simulink model "r2_b16a4x64f"  (R2012b)
settings: Solver=VariableStepDiscrete  SolverMode=SingleTasking  StartTime=0.0  StopTime=1  RelTol=1e-3
undefined symbols (not defined in the file): fft_stages, n_bits_ants, n_bits_xengs
libraries: xbsIndex_r4 x26846, casper_library_misc x230, xbsReplacements_r4 x24, casper_library_delays x8, xps_library x5, casper_library_communications x4
(part 51 of 227)

== system r2_b16a4x64f/sys2/tl_reord_flags ==
  note: Time has come
  note: Pulse as
      | value
      | changes
  note: Load value when armed
      | and time has come
      | or loading now
  rst : Inport
  current_time : Inport  Port=2
  load_value : Inport  Port=3
  en : Inport  Port=4
  misci : Inport  Port=5
  Assert : xbsIndex_r4/Assert  assert_type=on  type_source=Explicitly  gui_display_data_type=Fixed-point  arith_type=Boolean  n_bits=16  bin_pt=14  preci_type=Single  exp_width=8  frac_width=24  assert_rate=on  rate_source=Explicitly  period=1  output_port=on  block_type=assert
      settings: block_version=11.4
  Concat9 : xbsIndex_r4/Concat  num_inputs=2  dbl_ovrd=off  block_type=concat
      settings: block_version=10.1.3
  Constant29 : Constant  Value=20
  Delay{1..10,13..14,17..20,25..27} (19 alike) : xbsIndex_r4/Delay  rst=off  infoeditControl=Selection of Reset will increase slice count due to use of real FFs and instead of SRLs  en=off  latency=1  dbl_ovrd=off  reg_retiming=on  block_type=delay
  Delay{11..12,15..16} (4 alike) : xbsIndex_r4/Delay  rst=off  infoeditControl=Selection of Reset will increase slice count due to use of real FFs and instead of SRLs  en=on  latency=1  dbl_ovrd=off  reg_retiming=on  block_type=delay
  Inverter : xbsIndex_r4/Inverter  en=off  latency=0  dbl_ovrd=off  block_type=inv
      settings: block_version=11.4
  Logical1 : xbsIndex_r4/Logical  logical_function=AND  inputs=3  en=off  latency=0  precision=Full  arith_type=Unsigned  n_bits=16  bin_pt=0  align_bp=on  dbl_ovrd=off  block_type=logical
  Logical2 : xbsIndex_r4/Logical  logical_function=OR  inputs=2  en=off  latency=1  precision=Full  arith_type=Unsigned  n_bits=16  bin_pt=0  align_bp=on  dbl_ovrd=off  block_type=logical
  Logical3 : xbsIndex_r4/Logical  logical_function=AND  inputs=2  en=off  latency=0  precision=Full  arith_type=Unsigned  n_bits=16  bin_pt=0  align_bp=on  dbl_ovrd=off  block_type=logical
  Logical4 : xbsIndex_r4/Logical  logical_function=AND  inputs=2  en=off  latency=0  precision=Full  arith_type=Unsigned  n_bits=16  bin_pt=0  align_bp=on  dbl_ovrd=off  block_type=logical
  Logical5 : xbsIndex_r4/Logical  logical_function=OR  inputs=2  en=off  latency=0  precision=Full  arith_type=Unsigned  n_bits=16  bin_pt=0  align_bp=on  dbl_ovrd=off  block_type=logical
  Relational : xbsIndex_r4/Relational  mode=a=b  en=off  latency=1  dbl_ovrd=off  block_type=relational
      settings: block_version=10.1.3
  Slice1 : xbsIndex_r4/Slice  nbits=n_bits_time - n_bits_offset  boolean_output=off  mode=Lower Bit Location + Width  bit1=0  base1=MSB of Input  bit0=n_bits_offset  base0=LSB of Input  dbl_ovrd=off  block_type=slice
  Slice2 : xbsIndex_r4/Slice  nbits=n_bits_time - n_bits_offset  boolean_output=off  mode=Lower Bit Location + Width  bit1=0  base1=MSB of Input  bit0=n_bits_offset  base0=LSB of Input  dbl_ovrd=off  block_type=slice
  control : Subsystem  Tag=xps:sw_reg  AncestorBlock=xps_library/software register  mask(swreg){mode=one value, io_dir=From Processor, io_delay=0, sample_period=1, names=load_time_lsw, bitwidths=32, arith_types=0, bin_pts=0, sim_port=on, show_format=off}
      mask prompts: io_dir "I/O direction"; io_delay "I/O delay"; sample_period "Sample period"; names "Name:"; bitwidths "Bitwidth:"; arith_types "Type (ufix=0, fix=1, bool=2):"; bin_pts "Binary pt:"; sim_port "Provide sim input/output?"; show_format "Print format string?"
      mask init:
      | swreg_init(gcb)
      settings: AttributesFormatString=1input
      mask TypeOptions mode: one value | fields of equal size | fields of arbitrary size
      mask Callback mode: swreg_cb(gcb);
      mask TypeOptions io_dir: To Processor | From Processor
      mask Callback io_dir:
      | mask_enables = get_param(gcb, 'MaskEnables');
      | mask_names = get_param(gcb, 'MaskNames');
      | if strcmp(get_param(gcb, 'io_dir'), 'To Processor'),
      |     mask_enables{ismember(mask_names, 'sample_period')} = 'off';
      | else
      |     mask_enables{ismember(mask_names, 'sample_period')} = 'on';
      | end
      | set_param(gcb, 'MaskEnables', mask_enables);
      mask Callback bitwidths:
      | swreg_maskcheck(gcb);
      | % blk = gcb;
      | % mode = get_param(blk, 'mode');
      | % current_widths = eval(get_param(blk, 'bitwidths'));
      | % if (strcmp(mode, 'one value') || strcmp(mode, 'fields of equal size')) && (length(current_widths) > 1),
      | %     error('Only one width may be specified for this mode.');
      | % elseif strcmp(mode, 'fields of arbitrary size')
      | %     current_names = textscan(strtrim(strrep(strrep(get_param(blk, 'names'), ']', ''), '[', '')), '%s');
      | %     current_names = current_names{1};
      | %     numios = length(current_names);
      | %     if length(current_widths) ~= numios,
      | %         error('%d field names specified, but %d widths?', numios, length(current_widths));
      | %     end
      | % end
      | % total_width = 0;
      | % for ctr = 1 : length(current_widths),
      | %     total_width = total_width + current_widths(ctr);
      | % end
      | % if total_width > 32,
      | %     error('Total width must be 32 or less, set to %d.', total_width);
      | % end
      mask Callback arith_types:
      | [numios, ~, ~, ~, current_types] = swreg_maskcheck(gcb);
      | % blk = gcb;
      | % mode = get_param(blk, 'mode');
      | % current_types = eval(get_param(blk, 'arith_types'));
      | % numios = length(current_types);
      | % if (strcmp(mode, 'one value') || strcmp(mode, 'fields of equal size')) && (length(current_types) > 1),
      | %     error('Only one type may be specified for this mode.');
      | % elseif strcmp(mode, 'fields of arbitrary size')
      | %     current_names = textscan(strtrim(strrep(strrep(get_param(blk, 'names'), ']', ''), '[', '')), '%s');
      | %     current_names = current_names{1};
      | %     numios = length(current_names);
      | %     if length(current_types) ~= numios,
      | %         error('%d field names specified, but %d types?', numios, length(current_types));
      | %     end
      | % end
      | problem = 0;
      | for ctr = 1 : numios,
      |     t = current_types(ctr);
      |     if (t < 0) || (t > 2),
      |         problem = t;
      |         ctr = numios + 1;
      |     end
      | end
      | if problem ~= 0,
      |     error('Type cannot be %i, must be 0, 1 or 2.', problem);
      | end
      mask Callback bin_pts:
      | swreg_maskcheck(gcb);
      | % blk = gcb;
      | % mode = get_param(blk, 'mode');
      | % current_bins = eval(get_param(blk, 'bin_pts'));
      | % if (strcmp(mode, 'one value') || strcmp(mode, 'fields of equal size')) && (length(current_bins) > 1),
      | %     error('Only one binary pt may be specified for this mode.');
      | % elseif strcmp(mode, 'fields of arbitrary size')
      | %     current_names = textscan(strtrim(strrep(strrep(get_param(blk, 'names'), ']', ''), '[', '')), '%s');
      | %     current_names = current_names{1};
      | %     numios = length(current_names);
      | %     if length(current_bins) ~= numios,
      | %         error('%d field names specified, but %d binary pts?', numios, length(current_bins));
      | %     end
      | % end
  control0 : Subsystem  Tag=xps:sw_reg  AncestorBlock=xps_library/software register  mask(swreg){mode=fields of arbitrary size, io_dir=From Processor, io_delay=0, sample_period=1, names=[arm load_immediate load_time_msw], bitwidths=[1 1 16], arith_types=[2 2 0], bin_pts=[0 0 0], sim_port=off, show_format=off}
      mask prompts: io_dir "I/O direction"; io_delay "I/O delay"; sample_period "Sample period"; names "Names [msb ... lsb]:"; bitwidths "Bitwidths [msb ... lsb]:"; arith_types "Types (ufix=0, fix=1, bool=2) [msb ... lsb]:"; bin_pts "Binary pts [msb ... lsb]:"; sim_port "Provide sim input/output?"; show_format "Print format string?"
      mask init:
      | swreg_init(gcb)
      settings: AttributesFormatString=3 inputs
      mask TypeOptions mode: one value | fields of equal size | fields of arbitrary size
      mask Callback mode: swreg_cb(gcb);
      mask TypeOptions io_dir: To Processor | From Processor
      mask Callback io_dir:
      | mask_enables = get_param(gcb, 'MaskEnables');
      | mask_names = get_param(gcb, 'MaskNames');
      | if strcmp(get_param(gcb, 'io_dir'), 'To Processor'),
      |     mask_enables{ismember(mask_names, 'sample_period')} = 'off';
      | else
      |     mask_enables{ismember(mask_names, 'sample_period')} = 'on';
      | end
      | set_param(gcb, 'MaskEnables', mask_enables);
      mask Callback bitwidths:
      | swreg_maskcheck(gcb);
      | % blk = gcb;
      | % mode = get_param(blk, 'mode');
      | % current_widths = eval(get_param(blk, 'bitwidths'));
      | % if (strcmp(mode, 'one value') || strcmp(mode, 'fields of equal size')) && (length(current_widths) > 1),
      | %     error('Only one width may be specified for this mode.');
      | % elseif strcmp(mode, 'fields of arbitrary size')
      | %     current_names = textscan(strtrim(strrep(strrep(get_param(blk, 'names'), ']', ''), '[', '')), '%s');
      | %     current_names = current_names{1};
      | %     numios = length(current_names);
      | %     if length(current_widths) ~= numios,
      | %         error('%d field names specified, but %d widths?', numios, length(current_widths));
      | %     end
      | % end
      | % total_width = 0;
      | % for ctr = 1 : length(current_widths),
      | %     total_width = total_width + current_widths(ctr);
      | % end
      | % if total_width > 32,
      | %     error('Total width must be 32 or less, set to %d.', total_width);
      | % end
      mask Callback arith_types:
      | [numios, ~, ~, ~, current_types] = swreg_maskcheck(gcb);
      | % blk = gcb;
      | % mode = get_param(blk, 'mode');
      | % current_types = eval(get_param(blk, 'arith_types'));
      | % numios = length(current_types);
      | % if (strcmp(mode, 'one value') || strcmp(mode, 'fields of equal size')) && (length(current_types) > 1),
      | %     error('Only one type may be specified for this mode.');
      | % elseif strcmp(mode, 'fields of arbitrary size')
      | %     current_names = textscan(strtrim(strrep(strrep(get_param(blk, 'names'), ']', ''), '[', '')), '%s');
      | %     current_names = current_names{1};
      | %     numios = length(current_names);
      | %     if length(current_types) ~= numios,
      | %         error('%d field names specified, but %d types?', numios, length(current_types));
      | %     end
      | % end
      | problem = 0;
      | for ctr = 1 : numios,
      |     t = current_types(ctr);
      |     if (t < 0) || (t > 2),
      |         problem = t;
      |         ctr = numios + 1;
      |     end
      | end
      | if problem ~= 0,
      |     error('Type cannot be %i, must be 0, 1 or 2.', problem);
      | end
      mask Callback bin_pts:
      | swreg_maskcheck(gcb);
      | % blk = gcb;
      | % mode = get_param(blk, 'mode');
      | % current_bins = eval(get_param(blk, 'bin_pts'));
      | % if (strcmp(mode, 'one value') || strcmp(mode, 'fields of equal size')) && (length(current_bins) > 1),
      | %     error('Only one binary pt may be specified for this mode.');
      | % elseif strcmp(mode, 'fields of arbitrary size')
      | %     current_names = textscan(strtrim(strrep(strrep(get_param(blk, 'names'), ']', ''), '[', '')), '%s');
      | %     current_names = current_names{1};
      | %     numios = length(current_names);
      | %     if length(current_bins) ~= numios,
      | %         error('%d field names specified, but %d binary pts?', numios, length(current_bins));
      | %     end
      | % end
  count0 : xbsIndex_r4/Counter  cnt_type=Free Running  cnt_to=Inf  operation=Up  start_count=0  cnt_by_val=1  arith_type=Unsigned  n_bits=n_bits_counters  bin_pt=0  load_pin=off  rst=on  en=on  explicit_period=on  period=1  dbl_ovrd=off  use_behavioral_HDL=off  implementation=Fabric  block_type=counter
      settings: block_version=11.4
  count1 : xbsIndex_r4/Counter  cnt_type=Free Running  cnt_to=Inf  operation=Up  start_count=0  cnt_by_val=1  arith_type=Unsigned  n_bits=n_bits_counters  bin_pt=0  load_pin=off  rst=on  en=on  explicit_period=on  period=1  dbl_ovrd=off  use_behavioral_HDL=off  implementation=Fabric  block_type=counter
      settings: block_version=11.4
  edge_detect : Subsystem  AncestorBlock=casper_library_misc/edge_detect  mask(edge_detect){edge=Rising, polarity=Active High, x_in=[0 0.08 0.08 0.16 0.16 0.24 0.24 0.32 0.32 0.4], y_in=[-1 -1  1  1  1  1  1  1  1  1], x_out=[0.6 0.68 0.68 0.76 0.76 0.84 0.84 0.92 0.92 1], y_out=[-1 -1  1  1 -1 -1 -1 -1 -1 -1]}
      mask prompts: edge "Edge Type"; polarity "Output Polarity"; x_in "Input X Positions"; y_in "Input Y Positions"; x_out "Output X Positions"; y_out "Output Y Positions"
      mask help: Output is active for one-cycle after each edge of the specified type (i.e. rising, falling or both).
      mask init: same as r2_b16a4x64f/edge_detect
      settings: AttributesFormatString=|
      | rising edges
      | active high
      mask Help: Output is active for one-cycle after each edge of the specified type (i.e. rising, falling, or both).  Latency is zero.
      mask TypeOptions edge: Rising | Falling | Both
      mask TypeOptions polarity: Active High | Active Low
      mask Display:
      | plot(x_in_num,0.5+y_in_num*0.2);
      | plot(x_out_num,0.5+y_out_num*0.2);
  edge_detect1 : Subsystem  AncestorBlock=casper_library_misc/edge_detect  mask(edge_detect){edge=Rising, polarity=Active High, x_in=[0 0.08 0.08 0.16 0.16 0.24 0.24 0.32 0.32 0.4], y_in=[-1 -1  1  1  1  1  1  1  1  1], x_out=[0.6 0.68 0.68 0.76 0.76 0.84 0.84 0.92 0.92 1], y_out=[-1 -1  1  1 -1 -1 -1 -1 -1 -1]}
      mask prompts: edge "Edge Type"; polarity "Output Polarity"; x_in "Input X Positions"; y_in "Input Y Positions"; x_out "Output X Positions"; y_out "Output Y Positions"
      mask help: Output is active for one-cycle after each edge of the specified type (i.e. rising, falling or both).
      mask init: same as r2_b16a4x64f/edge_detect
      settings: AttributesFormatString=|
      | rising edges
      | active high
      mask Help: Output is active for one-cycle after each edge of the specified type (i.e. rising, falling, or both).  Latency is zero.
      mask TypeOptions edge: Rising | Falling | Both
      mask TypeOptions polarity: Active High | Active Low
      mask Display:
      | plot(x_in_num,0.5+y_in_num*0.2);
      | plot(x_out_num,0.5+y_out_num*0.2);
  pipeline : Subsystem  AncestorBlock=casper_library_delays/pipeline  mask(pipeline){latency=2}
      mask help:
      | An explicitly laid-out delay line to avoid mapping to SRL16s
      | for use in pipelining to help achieve timing closure.
      mask init:
      | pipeline_init(gcb,'latency',latency);
      settings: AttributesFormatString=Latency = %<latency>
      mask Display:
      | port_label('input', 1, 'd');
      | port_label('output', 1, 'q');
      | disp(['Z^-', num2str(latency)]);
  pipeline1 : Subsystem  AncestorBlock=casper_library_delays/pipeline  mask(pipeline){latency=2}
      mask help:
      | An explicitly laid-out delay line to avoid mapping to SRL16s
      | for use in pipelining to help achieve timing closure.
      mask init:
      | pipeline_init(gcb,'latency',latency);
      settings: AttributesFormatString=Latency = %<latency>
      mask Display:
      | port_label('input', 1, 'd');
      | port_label('output', 1, 'q');
      | disp(['Z^-', num2str(latency)]);
  pipeline2 : Subsystem  AncestorBlock=casper_library_delays/pipeline  mask(pipeline){latency=2}
      mask help:
      | An explicitly laid-out delay line to avoid mapping to SRL16s
      | for use in pipelining to help achieve timing closure.
      mask init:
      | pipeline_init(gcb,'latency',latency);
      settings: AttributesFormatString=Latency = %<latency>
      mask Display:
      | port_label('input', 1, 'd');
      | port_label('output', 1, 'q');
      | disp(['Z^-', num2str(latency)]);
  pipeline3 : Subsystem  AncestorBlock=casper_library_delays/pipeline  mask(pipeline){latency=2}
      mask help:
      | An explicitly laid-out delay line to avoid mapping to SRL16s
      | for use in pipelining to help achieve timing closure.
      mask init:
      | pipeline_init(gcb,'latency',latency);
      settings: AttributesFormatString=Latency = %<latency>
      mask Display:
      | port_label('input', 1, 'd');
      | port_label('output', 1, 'q');
      | disp(['Z^-', num2str(latency)]);
  pipeline4 : Subsystem  AncestorBlock=casper_library_delays/pipeline  mask(pipeline){latency=2}
      mask help:
      | An explicitly laid-out delay line to avoid mapping to SRL16s
      | for use in pipelining to help achieve timing closure.
      mask init:
      | pipeline_init(gcb,'latency',latency);
      settings: AttributesFormatString=Latency = %<latency>
      mask Display:
      | port_label('input', 1, 'd');
      | port_label('output', 1, 'q');
      | disp(['Z^-', num2str(latency)]);
  pipeline5 : Subsystem  AncestorBlock=casper_library_delays/pipeline  mask(pipeline){latency=2}
      mask help:
      | An explicitly laid-out delay line to avoid mapping to SRL16s
      | for use in pipelining to help achieve timing closure.
      mask init:
      | pipeline_init(gcb,'latency',latency);
      settings: AttributesFormatString=Latency = %<latency>
      mask Display:
      | port_label('input', 1, 'd');
      | port_label('output', 1, 'q');
      | disp(['Z^-', num2str(latency)]);
  status : Subsystem  Tag=xps:sw_reg  AncestorBlock=xps_library/software register  mask(swreg){mode=fields of arbitrary size, io_dir=To Processor, io_delay=1, sample_period=1, names=[armed arm_count load_count], bitwidths=[1 8 8], arith_types=[2 0 0], bin_pts=[0 0 0], sim_port=off, show_format=off}
      mask prompts: io_dir "I/O direction"; io_delay "I/O delay"; sample_period "Sample period"; names "Names [msb ... lsb]:"; bitwidths "Bitwidths [msb ... lsb]:"; arith_types "Types (ufix=0, fix=1, bool=2) [msb ... lsb]:"; bin_pts "Binary pts [msb ... lsb]:"; sim_port "Provide sim input/output?"; show_format "Print format string?"
      mask init:
      | swreg_init(gcb)
      settings: AttributesFormatString=3 outputs
      mask TypeOptions mode: one value | fields of equal size | fields of arbitrary size
      mask Callback mode: swreg_cb(gcb);
      mask TypeOptions io_dir: To Processor | From Processor
      mask Callback io_dir:
      | mask_enables = get_param(gcb, 'MaskEnables');
      | mask_names = get_param(gcb, 'MaskNames');
      | if strcmp(get_param(gcb, 'io_dir'), 'To Processor'),
      |     mask_enables{ismember(mask_names, 'sample_period')} = 'off';
      | else
      |     mask_enables{ismember(mask_names, 'sample_period')} = 'on';
      | end
      | set_param(gcb, 'MaskEnables', mask_enables);
      mask Callback bitwidths:
      | swreg_maskcheck(gcb);
      | % blk = gcb;
      | % mode = get_param(blk, 'mode');
      | % current_widths = eval(get_param(blk, 'bitwidths'));
      | % if (strcmp(mode, 'one value') || strcmp(mode, 'fields of equal size')) && (length(current_widths) > 1),
      | %     error('Only one width may be specified for this mode.');
      | % elseif strcmp(mode, 'fields of arbitrary size')
      | %     current_names = textscan(strtrim(strrep(strrep(get_param(blk, 'names'), ']', ''), '[', '')), '%s');
      | %     current_names = current_names{1};
      | %     numios = length(current_names);
      | %     if length(current_widths) ~= numios,
      | %         error('%d field names specified, but %d widths?', numios, length(current_widths));
      | %     end
      | % end
      | % total_width = 0;
      | % for ctr = 1 : length(current_widths),
      | %     total_width = total_width + current_widths(ctr);
      | % end
      | % if total_width > 32,
      | %     error('Total width must be 32 or less, set to %d.', total_width);
      | % end
      mask Callback arith_types:
      | [numios, ~, ~, ~, current_types] = swreg_maskcheck(gcb);
      | % blk = gcb;
      | % mode = get_param(blk, 'mode');
      | % current_types = eval(get_param(blk, 'arith_types'));
      | % numios = length(current_types);
      | % if (strcmp(mode, 'one value') || strcmp(mode, 'fields of equal size')) && (length(current_types) > 1),
      | %     error('Only one type may be specified for this mode.');
      | % elseif strcmp(mode, 'fields of arbitrary size')
      | %     current_names = textscan(strtrim(strrep(strrep(get_param(blk, 'names'), ']', ''), '[', '')), '%s');
      | %     current_names = current_names{1};
      | %     numios = length(current_names);
      | %     if length(current_types) ~= numios,
      | %         error('%d field names specified, but %d types?', numios, length(current_types));
      | %     end
      | % end
      | problem = 0;
      | for ctr = 1 : numios,
      |     t = current_types(ctr);
      |     if (t < 0) || (t > 2),
      |         problem = t;
      |         ctr = numios + 1;
      |     end
      | end
      | if problem ~= 0,
      |     error('Type cannot be %i, must be 0, 1 or 2.', problem);
      | end
      mask Callback bin_pts:
      | swreg_maskcheck(gcb);
      | % blk = gcb;
      | % mode = get_param(blk, 'mode');
      | % current_bins = eval(get_param(blk, 'bin_pts'));
      | % if (strcmp(mode, 'one value') || strcmp(mode, 'fields of equal size')) && (length(current_bins) > 1),
      | %     error('Only one binary pt may be specified for this mode.');
      | % elseif strcmp(mode, 'fields of arbitrary size')
      | %     current_names = textscan(strtrim(strrep(strrep(get_param(blk, 'names'), ']', ''), '[', '')), '%s');
      | %     current_names = current_names{1};
      | %     numios = length(current_names);
      | %     if length(current_bins) ~= numios,
      | %         error('%d field names specified, but %d binary pts?', numios, length(current_bins));
      | %     end
      | % end
  value : Outport
  enable : Outport  Port=2
  dvalid : Outport  Port=3
  time : Outport  Port=4
  misco : Outport  Port=5
  wires:
  Assert/1 -> Inverter/1, Logical4/1
  edge_detect/1(out) -> Delay2/1
  Slice2/1 -> Relational/1
  [load_time] -> Delay12/1
  Delay11/1 -> Delay15/1
  load_value/1 -> Delay11/1
  Delay12/1 -> Relational/2
  Delay27/1 -> enable/1
  Delay16/1 -> pipeline5/1(d), Assert/1, edge_detect/1(in), Logical1/1
  Delay15/1 -> value/1
  current_time/1 -> Slice2/1, Delay13/1
  [load_immediate] -> Delay25/1
  rst/1 -> [rst]
  [rst] -> count0/1
  [rst] -> count1/1
  Logical2/1 -> Logical1/2, Logical4/2
  Relational/1 -> Logical2/1
  Logical1/1 -> Delay3/1, Delay26/1, Delay1/1
  Inverter/1 -> Logical3/1, Delay16/1
  edge_detect1/1(out) -> Delay4/1
  Logical3/1 -> Logical5/1
  Logical4/1 -> Logical5/2
  Logical5/1 -> Delay16/2
  Delay2/1 -> count0/2
  Delay1/1 -> count1/2
  Delay3/1 -> Delay15/2
  [arm] -> edge_detect1/1(in)
  Delay4/1 -> Logical3/2, Delay12/2, Delay11/2
  Delay13/1 -> Delay17/1
  Delay14/1 -> Delay18/1
  count0/1 -> pipeline3/1(d)
  count1/1 -> pipeline4/1(d)
  Constant29/1 -> control/1(sim_1)
  control0/1(in_arm) -> pipeline/1(d)
  Concat9/1 -> pipeline2/1(d)
  control/1(in_load_time_lsw) -> Concat9/2
  control0/3(in_load_time_msw) -> Concat9/1
  control0/2(in_load_immediate) -> pipeline1/1(d)
  Delay17/1 -> Delay14/1
  Delay18/1 -> time/1
  Delay5/1 -> Delay6/1
  Delay7/1 -> Delay8/1
  en/1 -> Delay5/1
  Delay6/1 -> Delay7/1, Logical1/3
  Delay8/1 -> dvalid/1
  Delay9/1 -> Delay10/1
  Delay19/1 -> Delay20/1
  Delay10/1 -> Delay19/1
  misci/1 -> Delay9/1
  Delay20/1 -> misco/1
  Delay25/1 -> Logical2/2
  Delay26/1 -> Delay27/1
  pipeline/1(q) -> [arm]
  pipeline1/1(q) -> [load_immediate]
  pipeline2/1(q) -> Slice1/1
  Slice1/1 -> [load_time]
  pipeline5/1(q) -> status/1(out_armed)
  pipeline3/1(q) -> status/2(out_arm_count)
  pipeline4/1(q) -> status/3(out_load_count)

== system r2_b16a4x64f/sys2/vacc ==
  note: if flags go high at any point in the accumulation
      | they should be applied to the whole accumualtion
  rst : Inport
  arm : Inport  Port=2
  start_time : Inport  Port=3
  immediate : Inport  Port=4
  acc_len : Inport  Port=5
  sync_in : Inport  Port=6
  data_in : Inport  Port=7
  we : Inport  Port=8
  timestamp_in : Inport  Port=9
  flags_in : Inport  Port=10
  re : Inport  Port=11
  Concat10 : xbsIndex_r4/Concat  num_inputs=2  dbl_ovrd=off  block_type=concat
      settings: block_version=10.1.3
  Constant5 : xbsIndex_r4/Constant  const=0  gui_display_data_type=Fixed-point  arith_type=Unsigned  n_bits=4  bin_pt=0  preci_type=Single  exp_width=8  frac_width=24  explicit_period=on  period=1  equ=P=C  opselect=C  inp2=PCIN>>17  opr=+  inp1=P  carry=CIN  dbl_ovrd=off  block_type=constant
  Convert4 : xbsIndex_r4/Convert  gui_display_data_type=Fixed-point  arith_type=Unsigned  n_bits=16  bin_pt=0  float_type=Single  exp_bits=8  fraction_bits=24  quantization=Truncate  overflow=Wrap  en=off  latency=0  dbl_ovrd=off  pipeline=on  block_type=convert
      settings: block_version=11.4
  Convert5 : xbsIndex_r4/Convert  gui_display_data_type=Fixed-point  arith_type=Unsigned  n_bits=16  bin_pt=0  float_type=Single  exp_bits=8  fraction_bits=24  quantization=Truncate  overflow=Wrap  en=off  latency=0  dbl_ovrd=off  pipeline=on  block_type=convert
      settings: block_version=11.4
  Inverter : xbsIndex_r4/Inverter  en=off  latency=0  dbl_ovrd=off  block_type=inv
  Logical : xbsIndex_r4/Logical  logical_function=AND  inputs=2  en=off  latency=0  precision=Full  arith_type=Unsigned  n_bits=16  bin_pt=0  align_bp=on  dbl_ovrd=off  block_type=logical
  Logical2 : xbsIndex_r4/Logical  logical_function=AND  inputs=2  en=off  latency=0  precision=Full  arith_type=Unsigned  n_bits=16  bin_pt=0  align_bp=on  dbl_ovrd=off  block_type=logical
  Logical6 : xbsIndex_r4/Logical  logical_function=AND  inputs=2  en=off  latency=0  precision=Full  arith_type=Unsigned  n_bits=16  bin_pt=0  align_bp=on  dbl_ovrd=off  block_type=logical
  Register : xbsIndex_r4/Register  init=0  rst=on  en=on  dbl_ovrd=off  block_type=register
  Reinterpret1 : xbsIndex_r4/Reinterpret  force_arith_type=on  arith_type=Unsigned  force_bin_pt=on  bin_pt=0  block_type=reinterpret
      settings: block_version=10.1.3
  Terminator : Terminator
  bus_register : Subsystem  AncestorBlock=casper_library_bus/bus_register  mask(bus_register){reset=on, enable=on, cmplx=off, n_bits=n_bits_flags, misc=off}
      mask prompts: reset "reset port"; enable "enable port"; cmplx "complex data"; n_bits "input bit widths"; misc "misc support"
      mask help: Register components of bus
      mask init:
      | bus_register_init(gcb, ...
      |     'reset', reset, ...
      |     'enable', enable, ...
      |     'cmplx', cmplx, ...
      |     'n_bits', n_bits, ...
      |     'misc', misc);
  bus_relational : Subsystem  AncestorBlock=casper_library_bus/bus_relational  mask(bus_relational){n_bits_a=n_bits_flags, bin_pt_a=0, type_a=0, n_bits_b=n_bits_flags, bin_pt_b=0, type_b=0, en=off, misc=off, mode=a!=b, latency=0}
      mask prompts: n_bits_a "a input bit widths"; bin_pt_a "a input binary points"; type_a "a input type (Unsigned=0, Signed=1)"; n_bits_b "b input bit widths"; bin_pt_b "b input binary points"; type_b "b input type (Unsigned=0, Signed=1)"; en "en port"; misc "misc support"; mode "comparison:"
      mask help: Find the relational product of two busses
      mask init: same as r2_b16a4x64f/sys0/bus_relational
      mask TypeOptions mode: a=b | a!=b | a<b | a>b | a<=b | a>=b
  delay{1..3,5..6} (5 alike) : xbsIndex_r4/Delay  rst=off  infoeditControl=Selection of Reset will increase slice count due to use of real FFs and instead of SRLs  en=off  latency=2  dbl_ovrd=off  reg_retiming=on  block_type=delay
  delay10 : xbsIndex_r4/Delay  rst=off  infoeditControl=Selection of Reset will increase slice count due to use of real FFs and instead of SRLs  en=off  latency=1  dbl_ovrd=off  reg_retiming=on  block_type=delay
  delay4 : xbsIndex_r4/Delay  rst=off  infoeditControl=Selection of Reset will increase slice count due to use of real FFs and instead of SRLs  en=off  latency=1  dbl_ovrd=off  reg_retiming=on  block_type=delay
  flag_sampler : Subsystem  mask(sample_and_hold){period=(2^ants_bits)*(2^ants_bits +1) /2 * 8 * 2^(freq_bits-xeng_bits-n_inputs)}
      mask prompts: period "Sample period (clocks)"
      mask help: This block will sample an input signal at a user specified rate and hold the value on the output.
  mcnt_sampler : Subsystem  mask(sample_and_hold){period=(2^ants_bits)*(2^ants_bits +1) /2 * 8 * 2^(freq_bits-xeng_bits-n_inputs)}
      mask prompts: period "Sample period (clocks)"
      mask help: This block will sample an input signal at a user specified rate and hold the value on the output.
  qv : Subsystem  mask{vector_len=(2^ants_bits)*(2^ants_bits +1) /2 * 8 * 2^(freq_bits-xeng_bits-n_inputs), which_qdr=qdr2, n_bits=n_bits, n_inputs=n_inputs}
      mask prompts: vector_len "Vector length??(# cycles)"; which_qdr "Which QDR?"; n_bits "Data width (bits)"; n_inputs "Simultaneous inputs (2^?)"
      mask help:
      | A vector accumulator for medium length vectors designed for ROACH's QDR memory.
      |
      | Originally designed for the packetised correlator, this block accepts input data of type Fix_32_0. OOB_data_in provides an extra 4 bits that are accumulated seperately (originally designed to keep track of how many "bad" values in a vector were accumulated).
      |
      | Minimum vector length is 2 * burst_length.
      | Minimum burst length is 10 (recommended default is 2^4=16).
      |
      | The vector length does not need to be a multiple of the burst length.
      mask init: same as r2_b16a4x64f/sys0/vacc/qv
      settings: AttributesFormatString=Vector Length: 34816
      mask TypeOptions which_qdr: qdr0 | qdr1 | qdr2 | qdr3
  rst_replicate : Subsystem  AncestorBlock=casper_library_bus/bus_replicate  mask(bus_replicate){replication=length(n_bits_flags), latency=0, misc=off, implementation=behavioral}
      mask prompts: replication "replication factor"; misc "misc support"; implementation "delay implementation"
      mask help: Output bus formed by replicating input bus a number of times
      mask init:
      | bus_replicate_init(gcb, ...
      |     'replication', replication, ...
      |     'latency', latency, ...
      |     'implementation', implementation, ...
      |     'misc', misc);
      mask TypeOptions implementation: core | behavioral
  timestamp_reg1 : xbsIndex_r4/Register  init=0  rst=off  en=on  dbl_ovrd=off  block_type=register
  timestamp_reg2 : xbsIndex_r4/Register  init=0  rst=off  en=on  dbl_ovrd=off  block_type=register
  vacc_rst : Subsystem  mask{cnt_bits=8}
      mask prompts: cnt_bits "Bits in counters"
  zeros : Subsystem  AncestorBlock=casper_library_bus/bus_constant  mask(bus_constant){values=zeros(1, length(n_bits_flags)), n_bits=n_bits_flags, bin_pts=0, types=0}
      mask prompts: n_bits "bit widths"; bin_pts "binary points"; types "data type"
      mask help: Combine constants into a bus
      mask init:
      | bus_constant_init(gcb, ...
      |     'values', values, ...
      |     'n_bits', n_bits, ...
      |     'bin_pts', bin_pts, ...
      |     'types', types);
  new_acc : Outport
  data_out : Outport  Port=2
  oob_out : Outport  Port=3
  valid_out : Outport  Port=4
  pkt_rdy : Outport  Port=5
  rb_done : Outport  Port=6
  timestamp_out : Outport  Port=7
  flags_out : Outport  Port=8
  start_status : Outport  Port=9
  fifo_afull : Outport  Port=10
  error_out : Outport  Port=11
  error_flags : Outport  Port=12
  wires:
  [valid_out] -> Logical6/1
  [rb_done] -> Logical6/2
  start_time/1 -> vacc_rst/3(load_time)
  delay10/1 -> timestamp_reg2/2, Register/1, Register/3
  Logical6/1 -> delay10/1
  timestamp_reg1/1 -> timestamp_reg2/1
  delay4/1 -> timestamp_reg1/2
  [new_acc] -> delay4/1
  Concat10/1 -> start_status/1
  Inverter/1 -> qv/1(rst)
  timestamp_reg2/1 -> timestamp_out/1
  qv/7(fifo_afull) -> fifo_afull/1
  re/1 -> qv/7(ack_RB)
  qv/6(RB_done) -> [rb_done], rb_done/1
  we/1 -> delay3/1
  qv/5(error) -> error_out/1
  qv/4(valid) -> valid_out/1, [valid_out]
  data_in/1 -> delay2/1
  qv/3(oob_data_out) -> oob_out/1
  sync_in/1 -> delay1/1
  qv/2(data_out) -> data_out/1
  acc_len/1 -> qv/2(n_acum)
  qv/1(new_acc (ASYNC)) -> [new_acc], new_acc/1
  arm/1 -> vacc_rst/2(arm)
  rst/1 -> vacc_rst/1(rst)
  Constant5/1 -> qv/5(oob_data_in)
  Reinterpret1/1 -> qv/4(data_in)
  delay2/1 -> Reinterpret1/1
  delay3/1 -> qv/6(valid_data), mcnt_sampler/3(enable), flag_sampler/3(enable)
  delay5/1 -> mcnt_sampler/2(in)
  timestamp_in/1 -> vacc_rst/4(current_time), delay5/1
  vacc_rst/1(arm_count) -> Convert4/1
  vacc_rst/2(ld_count) -> Convert5/1
  Convert4/1 -> Concat10/1
  Convert5/1 -> Concat10/2
  Logical2/1 -> qv/3(sync)
  [vacc_en] -> Logical2/1, Inverter/1
  vacc_rst/3(enable) -> [vacc_en]
  immediate/1 -> vacc_rst/5(immediate)
  delay1/1 -> mcnt_sampler/1(sync), flag_sampler/1(sync), Logical2/2
  flags_in/1 -> delay6/1
  zeros/1(dout) -> bus_relational/1(a)
  flag_sampler/1(out) -> bus_relational/2(b), bus_register/1(din)
  bus_register/1(dout) -> flags_out/1
  qv/8(pkt_rdy) -> pkt_rdy/1
  rst_replicate/1(out) -> bus_register/2(rst)
  delay6/1 -> flag_sampler/2(in)
  flag_sampler/2(sample_out) -> Logical/2, Register/2
  Register/1 -> Logical/1
  bus_relational/1(a!=b) -> bus_register/3(en)
  Logical/1 -> rst_replicate/1(in)
  qv/9(error_flags) -> error_flags/1
  mcnt_sampler/1(out) -> timestamp_reg1/1
  mcnt_sampler/2(sample_out) -> Terminator/1
